simulink subsystem "encodervelocidadZ"  (R2022b)
settings: Solver=VariableStepAuto  StartTime=0.0  StopTime=10.0  RelTol=1e-3
libraries: arduinosensorlib x2, simulink x1
settings Model: Creator=miriamfreiriasanjuan  LastModifiedBy=miriamfreiriasanjuan

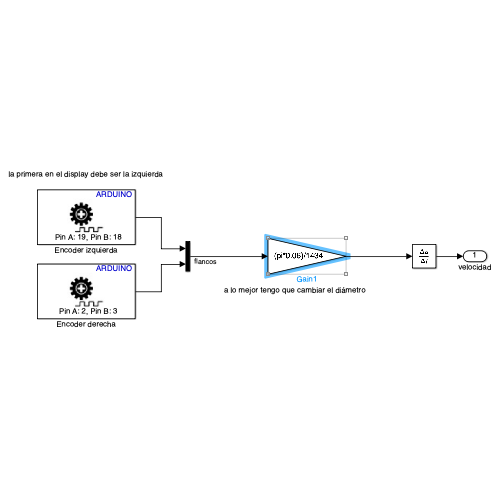
[thumbnail: Simulink's stored preview of the top-level diagram]
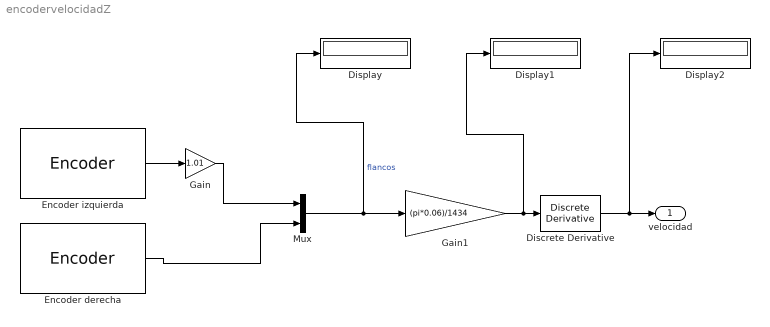
== system encodervelocidadZ ==
  Discrete Derivative : simulink/Discrete/Discrete Derivative  gainval=1.0  ICPrevScaledInput=0.0  OutMin=[]  OutMax=[]  OutDataType=fixdt(1, 16)  OutScaling=2^-10  DoSatur=off
  Display : Display
  Display1 : Display
  Display2 : Display
  Encoder derecha : arduinosensorlib/Encoder  InputA=2  InputB=3  Mode=No reset  SampleTime=-1
  Encoder izquierda : arduinosensorlib/Encoder  InputA=19  InputB=18  Mode=No reset  SampleTime=-1
  Gain : Gain  Gain=1.01  OutDataTypeStr=int32
  Gain1 : Gain  Gain=(pi*0.06)/1434  OutDataTypeStr=double
  Mux : Mux  Inputs=2
  velocidad : Outport
  wires:
  Discrete Derivative/1 -> Display2/1, velocidad/1
  Mux/1 -> Display/1, Gain1/1  "flancos"
  Gain1/1 -> Display1/1, Discrete Derivative/1
  Encoder derecha/1 -> Mux/2
  Encoder izquierda/1 -> Gain/1
  Gain/1 -> Mux/1
